simulink model "Main"  (R2025a)
settings: Solver=VariableStepAuto  StartTime=0.0  StopTime=inf  RelTol=1e-3
libraries: simulink x20, dspstat3 x10, simulink_extras x5, fuzblock x2
settings Model: Creator=felix  LastModifiedBy=lobakkang

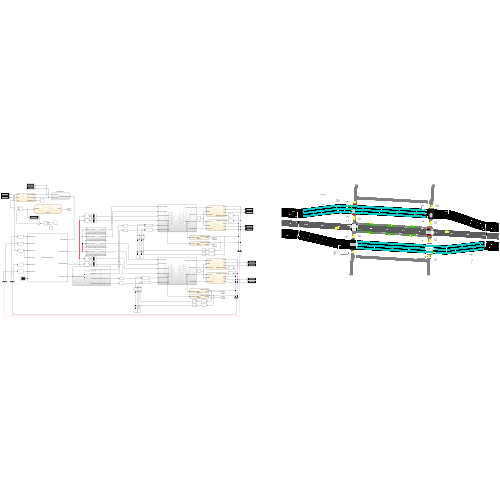
[thumbnail: Simulink's stored preview of the top-level diagram]
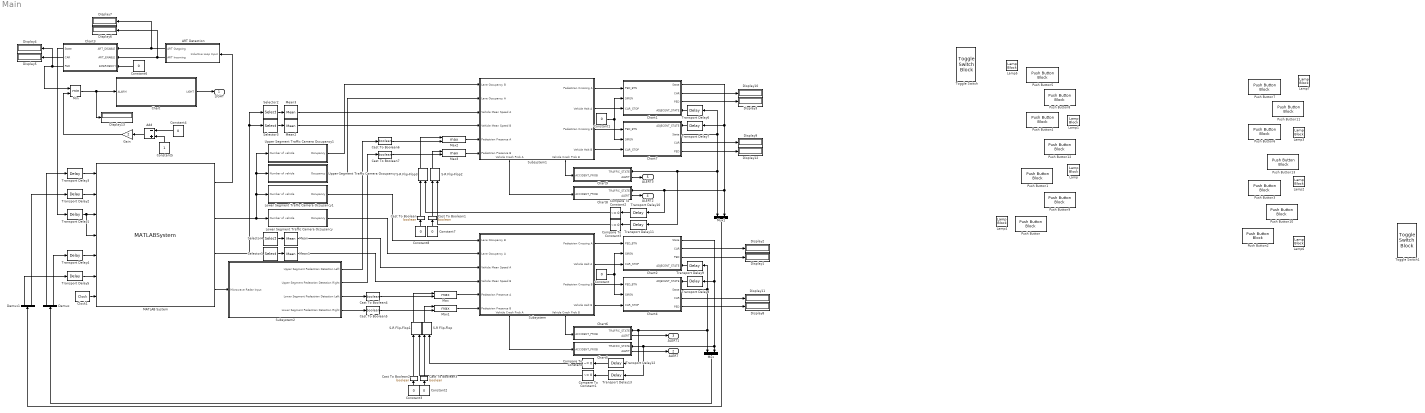
== system Main ==
  ART Detection : Subsystem
  Add : Sum  Inputs=-+
  Cast To Boolean{,1..7} (8 alike) : DataTypeConversion  OutDataTypeStr=boolean  SaturateOnIntegerOverflow=off  RndMeth=Floor
  Chart : Stateflow chart  TreatAsAtomicUnit=on
  Chart1 : Stateflow chart  TreatAsAtomicUnit=on
      settings: PortSchema="{\"entries\":[{\"content\":{\"sides\":[{\"content\":{\"connectorIds\":[\"In1\",\"In2\",\"In3\"]},\"type\":\"ConnectorPlacement.EquallySpacedRectSide\",\"uuid\":\"b25f2922-e8d8-447c-9fde-0a87dc56ab76\"},{\"content\":{\"connectorIds\":[\"Out1\",\"Out2\",\"Out3\",\"In4\"],\"side\":\"RIGHT\"},\"type\":\"ConnectorPlacement.EquallySpacedRectSide\",\"uuid\":\"421829cc-50ad-4948-b5ba-34d182ed9193\"},{\"content\":{\"side\":\"TOP\"},\"type\":\"ConnectorPlacement.EquallySpacedRectSide\",\"uuid\":\"15dcb3c0-9d0d-47c7-88ca-53369059b405\"},{\"content\":{\"side\":\"BOTTOM\"},\"type\":\"ConnectorPlacement.EquallySpacedRectSide\",\"uuid\":\"532ca745-839c-4cfc-92a4-9e4b119a98df\"}]},\"type\":\"ConnectorPlacement.EquallySpacedConnector\",\"uuid\":\"2a59643b-3d5f-42d6-a12d-4f5ba76c6b25\"}],\"packageUris\":[\"http://schema.mathworks.com/mf0/Connector/R2020b\"],\"version\":\"1.0\"}"
  Chart2 : Stateflow chart  TreatAsAtomicUnit=on
      settings: PortSchema="{\"entries\":[{\"content\":{\"sides\":[{\"content\":{\"connectorIds\":[\"In1\",\"In2\",\"In3\"]},\"type\":\"ConnectorPlacement.EquallySpacedRectSide\",\"uuid\":\"b25f2922-e8d8-447c-9fde-0a87dc56ab76\"},{\"content\":{\"connectorIds\":[\"Out1\",\"Out2\",\"Out3\",\"In4\"],\"side\":\"RIGHT\"},\"type\":\"ConnectorPlacement.EquallySpacedRectSide\",\"uuid\":\"421829cc-50ad-4948-b5ba-34d182ed9193\"},{\"content\":{\"side\":\"TOP\"},\"type\":\"ConnectorPlacement.EquallySpacedRectSide\",\"uuid\":\"15dcb3c0-9d0d-47c7-88ca-53369059b405\"},{\"content\":{\"side\":\"BOTTOM\"},\"type\":\"ConnectorPlacement.EquallySpacedRectSide\",\"uuid\":\"532ca745-839c-4cfc-92a4-9e4b119a98df\"}]},\"type\":\"ConnectorPlacement.EquallySpacedConnector\",\"uuid\":\"2a59643b-3d5f-42d6-a12d-4f5ba76c6b25\"}],\"packageUris\":[\"http://schema.mathworks.com/mf0/Connector/R2020b\"],\"version\":\"1.0\"}"
  Chart3 : Stateflow chart  TreatAsAtomicUnit=on
  Chart4 : Stateflow chart  TreatAsAtomicUnit=on
      settings: PortSchema="{\"entries\":[{\"content\":{\"sides\":[{\"content\":{\"connectorIds\":[\"In1\",\"In2\",\"In3\"]},\"type\":\"ConnectorPlacement.EquallySpacedRectSide\",\"uuid\":\"b25f2922-e8d8-447c-9fde-0a87dc56ab76\"},{\"content\":{\"connectorIds\":[\"In4\",\"Out1\",\"Out2\",\"Out3\"],\"side\":\"RIGHT\"},\"type\":\"ConnectorPlacement.EquallySpacedRectSide\",\"uuid\":\"421829cc-50ad-4948-b5ba-34d182ed9193\"},{\"content\":{\"side\":\"TOP\"},\"type\":\"ConnectorPlacement.EquallySpacedRectSide\",\"uuid\":\"15dcb3c0-9d0d-47c7-88ca-53369059b405\"},{\"content\":{\"side\":\"BOTTOM\"},\"type\":\"ConnectorPlacement.EquallySpacedRectSide\",\"uuid\":\"532ca745-839c-4cfc-92a4-9e4b119a98df\"}]},\"type\":\"ConnectorPlacement.EquallySpacedConnector\",\"uuid\":\"2a59643b-3d5f-42d6-a12d-4f5ba76c6b25\"}],\"packageUris\":[\"http://schema.mathworks.com/mf0/Connector/R2020b\"],\"version\":\"1.0\"}"
  Chart5 : Stateflow chart  TreatAsAtomicUnit=on
      settings: PortSchema="{\"entries\":[{\"content\":{\"sides\":[{\"content\":{\"connectorIds\":[\"In1\"]},\"type\":\"ConnectorPlacement.EquallySpacedRectSide\",\"uuid\":\"608d7dae-9529-4484-b16a-7c3c809a7af0\"},{\"content\":{\"connectorIds\":[\"In2\",\"Out1\"],\"side\":\"RIGHT\"},\"type\":\"ConnectorPlacement.EquallySpacedRectSide\",\"uuid\":\"13cec86d-a091-47ca-8c4c-06ad3ff59467\"},{\"content\":{\"side\":\"TOP\"},\"type\":\"ConnectorPlacement.EquallySpacedRectSide\",\"uuid\":\"91446a41-bf15-447e-8e76-a1311523585e\"}]},\"type\":\"ConnectorPlacement.EquallySpacedConnector\",\"uuid\":\"2a449cf7-a9fb-45d9-8ab4-45d23c1a1ddf\"}],\"packageUris\":[\"http://schema.mathworks.com/mf0/Connector/R2020b\"],\"version\":\"1.0\"}"
  Chart6 : Stateflow chart  TreatAsAtomicUnit=on
      settings: PortSchema="{\"entries\":[{\"content\":{\"sides\":[{\"content\":{\"connectorIds\":[\"In1\"]},\"type\":\"ConnectorPlacement.EquallySpacedRectSide\",\"uuid\":\"608d7dae-9529-4484-b16a-7c3c809a7af0\"},{\"content\":{\"connectorIds\":[\"In2\",\"Out1\"],\"side\":\"RIGHT\"},\"type\":\"ConnectorPlacement.EquallySpacedRectSide\",\"uuid\":\"13cec86d-a091-47ca-8c4c-06ad3ff59467\"},{\"content\":{\"side\":\"TOP\"},\"type\":\"ConnectorPlacement.EquallySpacedRectSide\",\"uuid\":\"91446a41-bf15-447e-8e76-a1311523585e\"}]},\"type\":\"ConnectorPlacement.EquallySpacedConnector\",\"uuid\":\"2a449cf7-a9fb-45d9-8ab4-45d23c1a1ddf\"}],\"packageUris\":[\"http://schema.mathworks.com/mf0/Connector/R2020b\"],\"version\":\"1.0\"}"
  Chart7 : Stateflow chart  TreatAsAtomicUnit=on
      settings: PortSchema="{\"entries\":[{\"content\":{\"sides\":[{\"content\":{\"connectorIds\":[\"In1\",\"In2\",\"In3\"]},\"type\":\"ConnectorPlacement.EquallySpacedRectSide\",\"uuid\":\"b25f2922-e8d8-447c-9fde-0a87dc56ab76\"},{\"content\":{\"connectorIds\":[\"In4\",\"Out1\",\"Out2\",\"Out3\"],\"side\":\"RIGHT\"},\"type\":\"ConnectorPlacement.EquallySpacedRectSide\",\"uuid\":\"421829cc-50ad-4948-b5ba-34d182ed9193\"},{\"content\":{\"side\":\"TOP\"},\"type\":\"ConnectorPlacement.EquallySpacedRectSide\",\"uuid\":\"15dcb3c0-9d0d-47c7-88ca-53369059b405\"},{\"content\":{\"side\":\"BOTTOM\"},\"type\":\"ConnectorPlacement.EquallySpacedRectSide\",\"uuid\":\"532ca745-839c-4cfc-92a4-9e4b119a98df\"}]},\"type\":\"ConnectorPlacement.EquallySpacedConnector\",\"uuid\":\"2a59643b-3d5f-42d6-a12d-4f5ba76c6b25\"}],\"packageUris\":[\"http://schema.mathworks.com/mf0/Connector/R2020b\"],\"version\":\"1.0\"}"
  Chart8 : Stateflow chart  TreatAsAtomicUnit=on
      settings: PortSchema="{\"entries\":[{\"content\":{\"sides\":[{\"content\":{\"connectorIds\":[\"In1\"]},\"type\":\"ConnectorPlacement.EquallySpacedRectSide\",\"uuid\":\"608d7dae-9529-4484-b16a-7c3c809a7af0\"},{\"content\":{\"connectorIds\":[\"In2\",\"Out1\"],\"side\":\"RIGHT\"},\"type\":\"ConnectorPlacement.EquallySpacedRectSide\",\"uuid\":\"13cec86d-a091-47ca-8c4c-06ad3ff59467\"},{\"content\":{\"side\":\"TOP\"},\"type\":\"ConnectorPlacement.EquallySpacedRectSide\",\"uuid\":\"91446a41-bf15-447e-8e76-a1311523585e\"}]},\"type\":\"ConnectorPlacement.EquallySpacedConnector\",\"uuid\":\"2a449cf7-a9fb-45d9-8ab4-45d23c1a1ddf\"}],\"packageUris\":[\"http://schema.mathworks.com/mf0/Connector/R2020b\"],\"version\":\"1.0\"}"
  Chart9 : Stateflow chart  TreatAsAtomicUnit=on
      settings: PortSchema="{\"entries\":[{\"content\":{\"sides\":[{\"content\":{\"connectorIds\":[\"In1\"]},\"type\":\"ConnectorPlacement.EquallySpacedRectSide\",\"uuid\":\"608d7dae-9529-4484-b16a-7c3c809a7af0\"},{\"content\":{\"connectorIds\":[\"In2\",\"Out1\"],\"side\":\"RIGHT\"},\"type\":\"ConnectorPlacement.EquallySpacedRectSide\",\"uuid\":\"13cec86d-a091-47ca-8c4c-06ad3ff59467\"},{\"content\":{\"side\":\"TOP\"},\"type\":\"ConnectorPlacement.EquallySpacedRectSide\",\"uuid\":\"91446a41-bf15-447e-8e76-a1311523585e\"}]},\"type\":\"ConnectorPlacement.EquallySpacedConnector\",\"uuid\":\"2a449cf7-a9fb-45d9-8ab4-45d23c1a1ddf\"}],\"packageUris\":[\"http://schema.mathworks.com/mf0/Connector/R2020b\"],\"version\":\"1.0\"}"
  Clock1 : simulink_extras/Flip Flops/Clock  period=1
  Compare To Constant{,1..3} (4 alike) : simulink/Logic and Bit Operations/Compare To Constant  relop=~=  const=0  OutDataTypeStr=boolean
  Constant{,1..4,6..8} (8 alike) : Constant  Value=0
  Constant5 : Constant
  Demux : Demux  Outputs=2
  Demux1 : Demux  Outputs=2
  Display{1..13} (13 alike) : Display
  Gain : Gain  Gain=2
  Lamp{,1..7} (8 alike) : LampBlock  LabelPosition=Hide  DefaultColor=[192.0, 192.0, 192.0]
  Lower Segment Traffic Camera Occupancy : Subsystem
  Lower Segment Traffic Camera Occupancy1 : Subsystem
  MATLAB System : MATLABSystem  System=TrafficSimulationSystem  Host=127.0.0.1  Port=55000  NumDetectors=4  NumInstantLoops=8  NumAreaDetectors=18  NumTrafficLights=6  SimulateUsing=Interpreted execution
      mask Type: TrafficSimulationSystem
  Max{,1..3} (4 alike) : MinMax  Function=max  Inputs=2
  Mean{,1..3} (4 alike) : dspstat3/Mean  run=off  InputProcessing=Columns as channels (frame based)  reset_popup=None  directionMode=Each column  dimension=1  roiEnable=off  roiType=Rectangles  roiPortion=Entire ROI  roiOutput=Individual statistics for each ROI  roiFlag=off  roundingMode=Floor  overflowMode=off  outputDataTypeStr=Inherit: Same as accumulator  outputMin=[]  outputMax=[]  outputLastDataTypeStr=Inherit: Same as accumulator
  Min : MinMax  Inputs=2
  Mux : Mux  Inputs=2
  Mux1 : Mux  Inputs=2
  Push Button{,1..5,7} (7 alike) : PushButtonBlock  IconOnColor=[0.0, 0.39215686274509803, 0.0]  IconOffColor=[0.0, 1.0, 0.0]  OffValue=0.000000
  Push Button{8..12} (5 alike) : PushButtonBlock  ButtonType=Latch  IconOnColor=[0.0, 0.39215686274509803, 0.0]  IconOffColor=[0.0, 1.0, 0.0]  OffValue=0.000000
  Push Button13 : PushButtonBlock  ButtonType=Latch  IconOnColor=[0.0, 0.39215686274509803, 0.0]  IconOffColor=[0.0, 1.0, 0.0]  OffValue=1.000000
  Push Button6 : PushButtonBlock  IconOnColor=[0.0, 0.39215686274509803, 0.0]  IconOffColor=[0.0, 1.0, 0.0]
  S-R Flip-Flop{,1..3} (4 alike) : simulink_extras/Flip Flops/S-R Flip-Flop  initial_condition=0
  Selector1 : Selector  IndexMode=Zero-based  InputPortWidth=18  IndexOptions=Index vector (dialog)  Indices=[6 7 8 9 10 11]  OutputSizes=1
  Selector2 : Selector  IndexMode=Zero-based  InputPortWidth=18  IndexOptions=Index vector (dialog)  Indices=[0 1 2 3 4 5]  OutputSizes=1
  Selector3 : Selector  IndexMode=Zero-based  InputPortWidth=18  IndexOptions=Index vector (dialog)  Indices=[12 13 15]  OutputSizes=1
  Selector4 : Selector  IndexMode=Zero-based  InputPortWidth=18  IndexOptions=Index vector (dialog)  Indices=[12 13 15]  OutputSizes=1
  Subsystem : Subsystem
      settings: PortSchema="{\"entries\":[{\"content\":{\"sides\":[{\"content\":{\"connectorIds\":[\"In1\",\"In2\",\"In3\",\"In4\",\"In5\",\"In6\"]},\"type\":\"ConnectorPlacement.EquallySpacedRectSide\",\"uuid\":\"53827b3a-c46a-4204-840d-e600012fe27f\"},{\"content\":{\"connectorIds\":[\"Out1\",\"Out2\",\"Out3\",\"Out4\"],\"side\":\"RIGHT\"},\"type\":\"ConnectorPlacement.EquallySpacedRectSide\",\"uuid\":\"cf707ced-ebab-43ca-9818-f6d8c721fe53\"},{\"content\":{\"side\":\"TOP\"},\"type\":\"ConnectorPlacement.EquallySpacedRectSide\",\"uuid\":\"16603e90-0a57-45b5-8379-ce405130782b\"},{\"content\":{\"connectorIds\":[\"Out5\",\"Out6\"],\"side\":\"BOTTOM\"},\"type\":\"ConnectorPlacement.EquallySpacedRectSide\",\"uuid\":\"f45158f6-4a74-4bd2-afbf-3c8c1bc11bef\"}]},\"type\":\"ConnectorPlacement.EquallySpacedConnector\",\"uuid\":\"52f23845-946f-443f-b18c-f1eea4db6dbd\"}],\"packageUris\":[\"http://schema.mathworks.com/mf0/Connector/R2020b\"],\"version\":\"1.0\"}"
  Subsystem1 : Subsystem
      settings: PortSchema="{\"entries\":[{\"content\":{\"sides\":[{\"content\":{\"connectorIds\":[\"In1\",\"In2\",\"In3\",\"In4\",\"In5\",\"In6\"]},\"type\":\"ConnectorPlacement.EquallySpacedRectSide\",\"uuid\":\"53827b3a-c46a-4204-840d-e600012fe27f\"},{\"content\":{\"connectorIds\":[\"Out1\",\"Out2\",\"Out3\",\"Out4\"],\"side\":\"RIGHT\"},\"type\":\"ConnectorPlacement.EquallySpacedRectSide\",\"uuid\":\"cf707ced-ebab-43ca-9818-f6d8c721fe53\"},{\"content\":{\"side\":\"TOP\"},\"type\":\"ConnectorPlacement.EquallySpacedRectSide\",\"uuid\":\"16603e90-0a57-45b5-8379-ce405130782b\"},{\"content\":{\"connectorIds\":[\"Out5\",\"Out6\"],\"side\":\"BOTTOM\"},\"type\":\"ConnectorPlacement.EquallySpacedRectSide\",\"uuid\":\"f45158f6-4a74-4bd2-afbf-3c8c1bc11bef\"}]},\"type\":\"ConnectorPlacement.EquallySpacedConnector\",\"uuid\":\"52f23845-946f-443f-b18c-f1eea4db6dbd\"}],\"packageUris\":[\"http://schema.mathworks.com/mf0/Connector/R2020b\"],\"version\":\"1.0\"}"
  Subsystem2 : Subsystem
  Toggle Switch : ToggleSwitchBlock
  Toggle Switch1 : ToggleSwitchBlock
  Transport Delay{1..13} (13 alike) : TransportDelay
  Upper Segment Traffic Camera Occupancy : Subsystem
  Upper Segment Traffic Camera Occupancy1 : Subsystem
  LIGHT : Outport
  ALERT : Outport  Port=2
  ALERT1 : Outport  Port=3
  ALERT2 : Outport  Port=4
  ALERT3 : Outport  Port=5
  wires:
  Transport Delay3/1 -> MATLAB System/1
  Transport Delay2/1 -> MATLAB System/2
  Chart3/3(PED) -> Display4/1, Min/1
  Chart3/2(CAR) -> Display5/1
  Transport Delay1/1 -> MATLAB System/4, MATLAB System/3
  Constant/1 -> Chart2/2(SIREN), Chart4/2(SIREN)
  Chart/1(LIGHT) -> LIGHT/1
  Min/1 -> Display13/1, Chart/1(ALARM)
  Gain/1 -> Min/2
  Add/1 -> Gain/1
  Constant4/1 -> Add/1
  Constant5/1 -> Add/2
  Constant6/1 -> Chart3/3(EMERGENCY)
  Clock1/1 -> MATLAB System/7
  Chart3/1(State) -> Transport Delay1/1
  MATLAB System/4 -> Subsystem2/1(Microwave Radar Input)
  ART Detection/2(ART Incoming) -> Chart3/2(ART_ENABLE), Display6/1
  ART Detection/1(ART Outgoing) -> Display7/1, Chart3/1(ART_DISABLE)
  MATLAB System/1 -> ART Detection/1(Inductive Loop Input)
  MATLAB System/3 -> Selector1/1, Selector2/1, Selector3/1, Selector4/1
  Selector4/1 -> Mean/1
  Selector1/1 -> Mean1/1
  Transport Delay4/1 -> MATLAB System/5
  Chart6/1(ALERT) -> ALERT1/1
  Lower Segment Traffic Camera Occupancy1/1(Occupancy) -> Subsystem/1(Lane Occupancy B)
  Lower Segment Traffic Camera Occupancy/1(Occupancy) -> Subsystem/2(Lane Occupancy A)
  Mean/1 -> Subsystem/3(Vehicle Mean Speed A)
  Mean1/1 -> Subsystem/4(Vehicle Mean Speed B)
  Subsystem/1(Pedestrian Crossing A) -> Chart2/1(PED_BTN)
  Subsystem/2(Vehicle Halt A) -> Chart2/3(CAR_STOP)
  Subsystem/3(Pedestrian Crossing B) -> Chart4/1(PED_BTN)
  Subsystem/4(Vehicle Halt B) -> Chart4/3(CAR_STOP)
  Subsystem/5(Vehicle Crash Prob A) -> Chart5/1(ACCIDENT_PROB)
  Subsystem/6(Vehicle Crash Prob B) -> Chart6/1(ACCIDENT_PROB)
  Transport Delay5/1 -> MATLAB System/6
  Demux/2 -> Transport Delay4/1
  Demux/1 -> Transport Delay3/1
  Chart4/1(State) -> Transport Delay12/1, Chart6/2(TRAFFIC_STATE), Mux/1, Transport Delay9/1
  Chart2/1(State) -> Transport Delay13/1, Chart5/2(TRAFFIC_STATE), Mux/2, Transport Delay8/1
  Chart1/1(State) -> Transport Delay7/1, Transport Delay10/1, Chart8/2(TRAFFIC_STATE), Mux1/2
  Chart7/1(State) -> Transport Delay11/1, Chart9/2(TRAFFIC_STATE), Mux1/1, Transport Delay6/1
  Subsystem1/6(Vehicle Crash Prob B) -> Chart9/1(ACCIDENT_PROB)
  Subsystem1/4(Vehicle Halt B) -> Chart7/3(CAR_STOP)
  Chart9/1(ALERT) -> ALERT3/1
  Subsystem1/2(Vehicle Halt A) -> Chart1/3(CAR_STOP)
  Subsystem1/3(Pedestrian Crossing B) -> Chart7/1(PED_BTN)
  Constant1/1 -> Chart1/2(SIREN), Chart7/2(SIREN)
  Chart1/2(CAR) -> Display10/1
  Subsystem1/5(Vehicle Crash Prob A) -> Chart8/1(ACCIDENT_PROB)
  Subsystem1/1(Pedestrian Crossing A) -> Chart1/1(PED_BTN)
  Chart8/1(ALERT) -> ALERT2/1
  Chart7/3(PED) -> Display12/1
  Chart1/3(PED) -> Display3/1
  Chart7/2(CAR) -> Display9/1
  Mux/1 -> Demux/1
  Mux1/1 -> Demux1/1
  MATLAB System/2 -> Lower Segment Traffic Camera Occupancy1/1(Number of vehicle), Upper Segment Traffic Camera Occupancy1/1(Number of vehicle), Upper Segment Traffic Camera Occupancy/1(Number of vehicle), Lower Segment Traffic Camera Occupancy/1(Number of vehicle)
  Upper Segment Traffic Camera Occupancy/1(Occupancy) -> Subsystem1/2(Lane Occupancy A)
  Upper Segment Traffic Camera Occupancy1/1(Occupancy) -> Subsystem1/1(Lane Occupancy B)
  Selector2/1 -> Mean3/1
  Selector3/1 -> Mean2/1
  Demux1/2 -> Transport Delay2/1
  Demux1/1 -> Transport Delay5/1
  Mean3/1 -> Subsystem1/3(Vehicle Mean Speed A)
  Mean2/1 -> Subsystem1/4(Vehicle Mean Speed B)
  Chart2/2(CAR) -> Display2/1
  Chart2/3(PED) -> Display1/1
  Chart4/2(CAR) -> Display11/1
  Chart4/3(PED) -> Display8/1
  Transport Delay6/1 -> Chart1/4(ADJECENT_STATE)
  Transport Delay7/1 -> Chart7/4(ADJECENT_STATE)
  Transport Delay8/1 -> Chart4/4(ADJECENT_STATE)
  Transport Delay9/1 -> Chart2/4(ADJECENT_STATE)
  Max1/1 -> Subsystem/6(Pedestrian Presence B)
  Max/1 -> Subsystem/5(Pedestrian Presence A)
  Subsystem2/3(Lower Segment Pedestrian Detection Left) -> Cast To Boolean4/1
  Subsystem2/4(Lower Segment Pedestrian Detection Right) -> Cast To Boolean5/1
  Max3/1 -> Subsystem1/6(Pedestrian Presence B)
  Subsystem2/2(Upper Segment Pedestrian Detection Right) -> Cast To Boolean7/1
  Max2/1 -> Subsystem1/5(Pedestrian Presence A)
  Subsystem2/1(Upper Segment Pedestrian Detection Left) -> Cast To Boolean6/1
  Chart5/1(ALERT) -> ALERT/1
  Constant2/1 -> Cast To Boolean3/1
  S-R Flip-Flop/1 -> Max1/1
  Constant3/1 -> Cast To Boolean2/1
  S-R Flip-Flop1/1 -> Max/1
  Compare To Constant/1 -> S-R Flip-Flop/2
  Compare To Constant1/1 -> S-R Flip-Flop1/2
  Constant7/1 -> Cast To Boolean1/1
  Constant8/1 -> Cast To Boolean/1
  S-R Flip-Flop2/1 -> Max3/1
  S-R Flip-Flop3/1 -> Max2/1
  Compare To Constant3/1 -> S-R Flip-Flop2/2
  Compare To Constant2/1 -> S-R Flip-Flop3/2
  Cast To Boolean/1 -> S-R Flip-Flop3/1
  Cast To Boolean1/1 -> S-R Flip-Flop2/1
  Cast To Boolean3/1 -> S-R Flip-Flop/1
  Cast To Boolean2/1 -> S-R Flip-Flop1/1
  Cast To Boolean4/1 -> Max/2
  Cast To Boolean5/1 -> Max1/2
  Cast To Boolean6/1 -> Max2/2
  Cast To Boolean7/1 -> Max3/2
  Transport Delay10/1 -> Compare To Constant2/1
  Transport Delay11/1 -> Compare To Constant3/1
  Transport Delay13/1 -> Compare To Constant1/1
  Transport Delay12/1 -> Compare To Constant/1

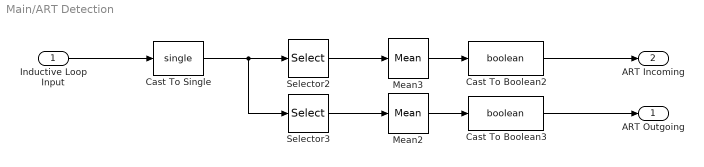
== system Main/ART Detection ==
  Inductive Loop Input : Inport
  Cast To Boolean2 : DataTypeConversion  OutDataTypeStr=boolean  SaturateOnIntegerOverflow=off  RndMeth=Floor
  Cast To Boolean3 : DataTypeConversion  OutDataTypeStr=boolean  SaturateOnIntegerOverflow=off  RndMeth=Floor
  Cast To Single : DataTypeConversion  OutDataTypeStr=single  SaturateOnIntegerOverflow=off  RndMeth=Floor
  Mean2 : dspstat3/Mean  run=off  InputProcessing=Columns as channels (frame based)  reset_popup=None  directionMode=Each column  dimension=1  roiEnable=off  roiType=Rectangles  roiPortion=Entire ROI  roiOutput=Individual statistics for each ROI  roiFlag=off  roundingMode=Floor  overflowMode=off  outputDataTypeStr=Inherit: Same as accumulator  outputMin=[]  outputMax=[]  outputLastDataTypeStr=Inherit: Same as accumulator
  Mean3 : dspstat3/Mean  run=off  InputProcessing=Columns as channels (frame based)  reset_popup=None  directionMode=Each column  dimension=1  roiEnable=off  roiType=Rectangles  roiPortion=Entire ROI  roiOutput=Individual statistics for each ROI  roiFlag=off  roundingMode=Floor  overflowMode=off  outputDataTypeStr=Inherit: Same as accumulator  outputMin=[]  outputMax=[]  outputLastDataTypeStr=Inherit: Same as accumulator
  Selector2 : Selector  InputPortWidth=4  IndexOptions=Index vector (dialog)  Indices=[3 2]  OutputSizes=1
  Selector3 : Selector  InputPortWidth=4  IndexOptions=Index vector (dialog)  Indices=[1 4]  OutputSizes=1
  ART Outgoing : Outport
  ART Incoming : Outport  Port=2
  wires:
  Mean2/1 -> Cast To Boolean3/1
  Mean3/1 -> Cast To Boolean2/1
  Cast To Single/1 -> Selector3/1, Selector2/1
  Selector3/1 -> Mean2/1
  Inductive Loop Input/1 -> Cast To Single/1
  Selector2/1 -> Mean3/1
  Cast To Boolean2/1 -> ART Incoming/1
  Cast To Boolean3/1 -> ART Outgoing/1

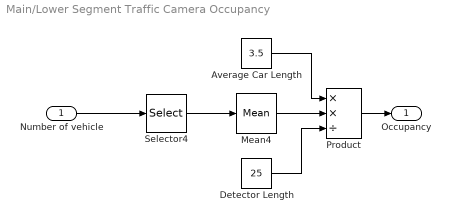
== system Main/Lower Segment Traffic Camera Occupancy ==
  Number of vehicle : Inport
  Average Car Length : Constant  Value=3.5
  Detector Length : Constant  Value=25
  Mean4 : dspstat3/Mean  run=off  InputProcessing=Columns as channels (frame based)  reset_popup=None  directionMode=Each column  dimension=1  roiEnable=off  roiType=Rectangles  roiPortion=Entire ROI  roiOutput=Individual statistics for each ROI  roiFlag=off  roundingMode=Floor  overflowMode=off  outputDataTypeStr=Inherit: Same as accumulator  outputMin=[]  outputMax=[]  outputLastDataTypeStr=Inherit: Same as accumulator
  Product : Product  Inputs=**/
  Selector4 : Selector  IndexMode=Zero-based  InputPortWidth=18  IndexOptions=Index vector (dialog)  Indices=[9 10 11 6 7 8]  OutputSizes=1
  Occupancy : Outport
  wires:
  Number of vehicle/1 -> Selector4/1
  Detector Length/1 -> Product/3
  Selector4/1 -> Mean4/1
  Mean4/1 -> Product/2
  Average Car Length/1 -> Product/1
  Product/1 -> Occupancy/1

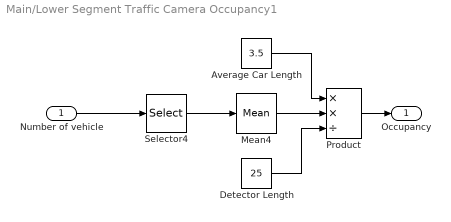
== system Main/Lower Segment Traffic Camera Occupancy1 ==
  Number of vehicle : Inport
  Average Car Length : Constant  Value=3.5
  Detector Length : Constant  Value=25
  Mean4 : dspstat3/Mean  run=off  InputProcessing=Columns as channels (frame based)  reset_popup=None  directionMode=Each column  dimension=1  roiEnable=off  roiType=Rectangles  roiPortion=Entire ROI  roiOutput=Individual statistics for each ROI  roiFlag=off  roundingMode=Floor  overflowMode=off  outputDataTypeStr=Inherit: Same as accumulator  outputMin=[]  outputMax=[]  outputLastDataTypeStr=Inherit: Same as accumulator
  Product : Product  Inputs=**/
  Selector4 : Selector  IndexMode=Zero-based  InputPortWidth=18  IndexOptions=Index vector (dialog)  Indices=[12 13 15]  OutputSizes=1
  Occupancy : Outport
  wires:
  Number of vehicle/1 -> Selector4/1
  Detector Length/1 -> Product/3
  Selector4/1 -> Mean4/1
  Mean4/1 -> Product/2
  Average Car Length/1 -> Product/1
  Product/1 -> Occupancy/1

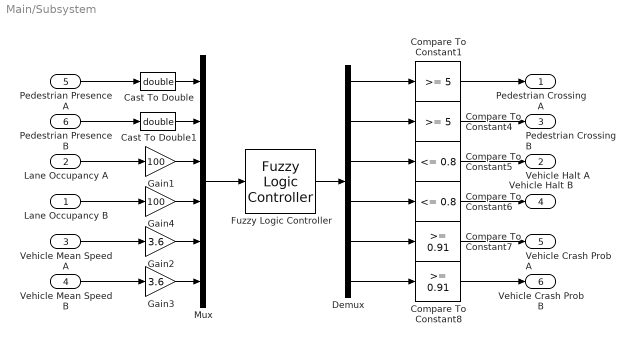
== system Main/Subsystem ==
  Lane Occupancy B : Inport
  Lane Occupancy A : Inport  Port=2
  Vehicle Mean Speed A : Inport  Port=3
  Vehicle Mean Speed B : Inport  Port=4
  Pedestrian Presence A : Inport  Port=5
  Pedestrian Presence B : Inport  Port=6
  Cast To Double : DataTypeConversion  OutDataTypeStr=double  SaturateOnIntegerOverflow=off  RndMeth=Floor
  Cast To Double1 : DataTypeConversion  OutDataTypeStr=double  SaturateOnIntegerOverflow=off  RndMeth=Floor
  Compare To Constant1 : simulink/Logic and Bit Operations/Compare To Constant  relop=>=  const=5  OutDataTypeStr=uint8
  Compare To Constant4 : simulink/Logic and Bit Operations/Compare To Constant  relop=>=  const=5  OutDataTypeStr=uint8
  Compare To Constant5 : simulink/Logic and Bit Operations/Compare To Constant  relop=<=  const=0.8  OutDataTypeStr=uint8
  Compare To Constant6 : simulink/Logic and Bit Operations/Compare To Constant  relop=<=  const=0.8  OutDataTypeStr=uint8
  Compare To Constant7 : simulink/Logic and Bit Operations/Compare To Constant  relop=>=  const=0.91  OutDataTypeStr=uint8
  Compare To Constant8 : simulink/Logic and Bit Operations/Compare To Constant  relop=>=  const=0.91  OutDataTypeStr=uint8
  Demux : Demux  Outputs=6
  Fuzzy Logic Controller : fuzblock/Fuzzy Logic  Controller  FIS='PedestrianController.fis'  OutputSampleNumber=101  DataType=double  UseLookupTable=off  NumBreakpoints=10  FuzzifiedInputs=off  RuleFiringStrengths=off  RuleOutputs=off  AggregatedOutputs=off  SimulateUsing=Code generation  OutOfRangeInputValueMessage=warning  NoRuleFiredMessage=warning  EmptyOutputFuzzySetMessage=warning
  Gain1 : Gain  Gain=100
  Gain2 : Gain  Gain=3.6
  Gain3 : Gain  Gain=3.6
  Gain4 : Gain  Gain=100
  Mux : Mux  Inputs=6
  Pedestrian Crossing A : Outport
  Vehicle Halt A : Outport  Port=2
  Pedestrian Crossing B : Outport  Port=3
  Vehicle Halt B : Outport  Port=4
  Vehicle Crash Prob A : Outport  Port=5
  Vehicle Crash Prob B : Outport  Port=6
  wires:
  Gain3/1 -> Mux/6
  Mux/1 -> Fuzzy Logic Controller/1
  Demux/1 -> Compare To Constant1/1
  Vehicle Mean Speed A/1 -> Gain2/1
  Demux/5 -> Compare To Constant7/1
  Fuzzy Logic Controller/1 -> Demux/1
  Demux/6 -> Compare To Constant8/1
  Cast To Double1/1 -> Mux/2
  Demux/4 -> Compare To Constant6/1
  Demux/3 -> Compare To Constant5/1
  Gain1/1 -> Mux/3
  Demux/2 -> Compare To Constant4/1
  Gain4/1 -> Mux/4
  Cast To Double/1 -> Mux/1
  Gain2/1 -> Mux/5
  Compare To Constant7/1 -> Vehicle Crash Prob A/1
  Pedestrian Presence B/1 -> Cast To Double1/1
  Pedestrian Presence A/1 -> Cast To Double/1
  Compare To Constant6/1 -> Vehicle Halt B/1
  Lane Occupancy A/1 -> Gain1/1
  Compare To Constant4/1 -> Pedestrian Crossing B/1
  Lane Occupancy B/1 -> Gain4/1
  Vehicle Mean Speed B/1 -> Gain3/1
  Compare To Constant8/1 -> Vehicle Crash Prob B/1
  Compare To Constant5/1 -> Vehicle Halt A/1
  Compare To Constant1/1 -> Pedestrian Crossing A/1

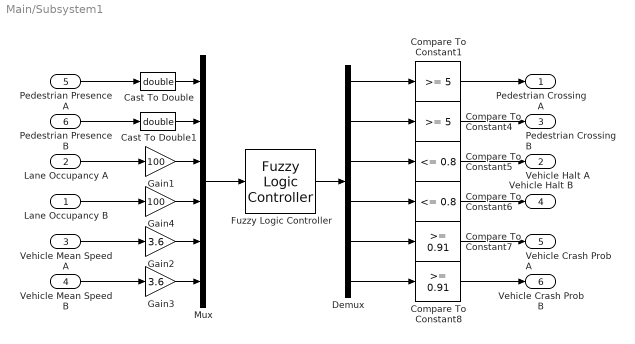
== system Main/Subsystem1 ==
  Lane Occupancy B : Inport
  Lane Occupancy A : Inport  Port=2
  Vehicle Mean Speed A : Inport  Port=3
  Vehicle Mean Speed B : Inport  Port=4
  Pedestrian Presence A : Inport  Port=5
  Pedestrian Presence B : Inport  Port=6
  Cast To Double : DataTypeConversion  OutDataTypeStr=double  SaturateOnIntegerOverflow=off  RndMeth=Floor
  Cast To Double1 : DataTypeConversion  OutDataTypeStr=double  SaturateOnIntegerOverflow=off  RndMeth=Floor
  Compare To Constant1 : simulink/Logic and Bit Operations/Compare To Constant  relop=>=  const=5  OutDataTypeStr=uint8
  Compare To Constant4 : simulink/Logic and Bit Operations/Compare To Constant  relop=>=  const=5  OutDataTypeStr=uint8
  Compare To Constant5 : simulink/Logic and Bit Operations/Compare To Constant  relop=<=  const=0.8  OutDataTypeStr=uint8
  Compare To Constant6 : simulink/Logic and Bit Operations/Compare To Constant  relop=<=  const=0.8  OutDataTypeStr=uint8
  Compare To Constant7 : simulink/Logic and Bit Operations/Compare To Constant  relop=>=  const=0.91  OutDataTypeStr=uint8
  Compare To Constant8 : simulink/Logic and Bit Operations/Compare To Constant  relop=>=  const=0.91  OutDataTypeStr=uint8
  Demux : Demux  Outputs=6
  Fuzzy Logic Controller : fuzblock/Fuzzy Logic  Controller  FIS='PedestrianController.fis'  OutputSampleNumber=101  DataType=double  UseLookupTable=off  NumBreakpoints=10  FuzzifiedInputs=off  RuleFiringStrengths=off  RuleOutputs=off  AggregatedOutputs=off  SimulateUsing=Code generation  OutOfRangeInputValueMessage=warning  NoRuleFiredMessage=warning  EmptyOutputFuzzySetMessage=warning
  Gain1 : Gain  Gain=100
  Gain2 : Gain  Gain=3.6
  Gain3 : Gain  Gain=3.6
  Gain4 : Gain  Gain=100
  Mux : Mux  Inputs=6
  Pedestrian Crossing A : Outport
  Vehicle Halt A : Outport  Port=2
  Pedestrian Crossing B : Outport  Port=3
  Vehicle Halt B : Outport  Port=4
  Vehicle Crash Prob A : Outport  Port=5
  Vehicle Crash Prob B : Outport  Port=6
  wires:
  Gain3/1 -> Mux/6
  Mux/1 -> Fuzzy Logic Controller/1
  Demux/1 -> Compare To Constant1/1
  Vehicle Mean Speed A/1 -> Gain2/1
  Demux/5 -> Compare To Constant7/1
  Fuzzy Logic Controller/1 -> Demux/1
  Demux/6 -> Compare To Constant8/1
  Cast To Double1/1 -> Mux/2
  Demux/4 -> Compare To Constant6/1
  Demux/3 -> Compare To Constant5/1
  Gain1/1 -> Mux/3
  Demux/2 -> Compare To Constant4/1
  Gain4/1 -> Mux/4
  Cast To Double/1 -> Mux/1
  Gain2/1 -> Mux/5
  Compare To Constant7/1 -> Vehicle Crash Prob A/1
  Pedestrian Presence B/1 -> Cast To Double1/1
  Pedestrian Presence A/1 -> Cast To Double/1
  Compare To Constant6/1 -> Vehicle Halt B/1
  Lane Occupancy A/1 -> Gain1/1
  Compare To Constant4/1 -> Pedestrian Crossing B/1
  Lane Occupancy B/1 -> Gain4/1
  Vehicle Mean Speed B/1 -> Gain3/1
  Compare To Constant8/1 -> Vehicle Crash Prob B/1
  Compare To Constant5/1 -> Vehicle Halt A/1
  Compare To Constant1/1 -> Pedestrian Crossing A/1

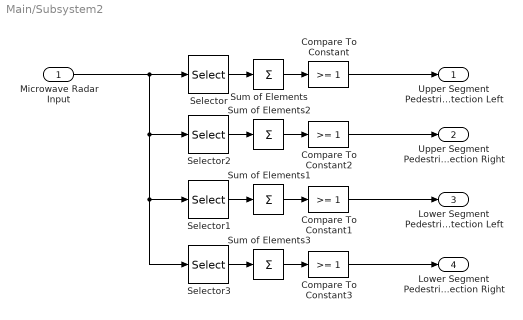
== system Main/Subsystem2 ==
  Microwave Radar Input : Inport
  Compare To Constant{,1..3} (4 alike) : simulink/Logic and Bit Operations/Compare To Constant  relop=>=  const=1  OutDataTypeStr=uint8
  Selector : Selector  InputPortWidth=8  IndexOptions=Index vector (dialog)  Indices=[6 7]  OutputSizes=1
  Selector1 : Selector  InputPortWidth=8  IndexOptions=Index vector (dialog)  Indices=[1 4]  OutputSizes=1
  Selector2 : Selector  InputPortWidth=8  IndexOptions=Index vector (dialog)  Indices=[5 8]  OutputSizes=1
  Selector3 : Selector  InputPortWidth=8  IndexOptions=Index vector (dialog)  Indices=[2 3]  OutputSizes=1
  Sum of Elements{,1..3} (4 alike) : Sum  Inputs=+
  Upper Segment Pedestrian Detection Left : Outport
  Upper Segment Pedestrian Detection Right : Outport  Port=2
  Lower Segment Pedestrian Detection Left : Outport  Port=3
  Lower Segment Pedestrian Detection Right : Outport  Port=4
  wires:
  Compare To Constant1/1 -> Lower Segment Pedestrian Detection Left/1
  Compare To Constant/1 -> Upper Segment Pedestrian Detection Left/1
  Sum of Elements/1 -> Compare To Constant/1
  Selector/1 -> Sum of Elements/1
  Selector1/1 -> Sum of Elements1/1
  Sum of Elements1/1 -> Compare To Constant1/1
  Compare To Constant2/1 -> Upper Segment Pedestrian Detection Right/1
  Selector2/1 -> Sum of Elements2/1
  Sum of Elements2/1 -> Compare To Constant2/1
  Selector3/1 -> Sum of Elements3/1
  Compare To Constant3/1 -> Lower Segment Pedestrian Detection Right/1
  Sum of Elements3/1 -> Compare To Constant3/1
  Microwave Radar Input/1 -> Selector/1, Selector2/1, Selector3/1, Selector1/1

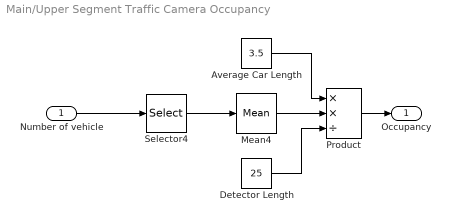
== system Main/Upper Segment Traffic Camera Occupancy ==
  Number of vehicle : Inport
  Average Car Length : Constant  Value=3.5
  Detector Length : Constant  Value=25
  Mean4 : dspstat3/Mean  run=off  InputProcessing=Columns as channels (frame based)  reset_popup=None  directionMode=Each column  dimension=1  roiEnable=off  roiType=Rectangles  roiPortion=Entire ROI  roiOutput=Individual statistics for each ROI  roiFlag=off  roundingMode=Floor  overflowMode=off  outputDataTypeStr=Inherit: Same as accumulator  outputMin=[]  outputMax=[]  outputLastDataTypeStr=Inherit: Same as accumulator
  Product : Product  Inputs=**/
  Selector4 : Selector  IndexMode=Zero-based  InputPortWidth=18  IndexOptions=Index vector (dialog)  Indices=[0 1 2 3 4 5]  OutputSizes=1
  Occupancy : Outport
  wires:
  Number of vehicle/1 -> Selector4/1
  Detector Length/1 -> Product/3
  Selector4/1 -> Mean4/1
  Mean4/1 -> Product/2
  Average Car Length/1 -> Product/1
  Product/1 -> Occupancy/1

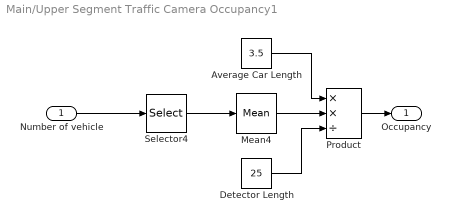
== system Main/Upper Segment Traffic Camera Occupancy1 ==
  Number of vehicle : Inport
  Average Car Length : Constant  Value=3.5
  Detector Length : Constant  Value=25
  Mean4 : dspstat3/Mean  run=off  InputProcessing=Columns as channels (frame based)  reset_popup=None  directionMode=Each column  dimension=1  roiEnable=off  roiType=Rectangles  roiPortion=Entire ROI  roiOutput=Individual statistics for each ROI  roiFlag=off  roundingMode=Floor  overflowMode=off  outputDataTypeStr=Inherit: Same as accumulator  outputMin=[]  outputMax=[]  outputLastDataTypeStr=Inherit: Same as accumulator
  Product : Product  Inputs=**/
  Selector4 : Selector  IndexMode=Zero-based  InputPortWidth=18  IndexOptions=Index vector (dialog)  Indices=[14 16 17]  OutputSizes=1
  Occupancy : Outport
  wires:
  Number of vehicle/1 -> Selector4/1
  Detector Length/1 -> Product/3
  Selector4/1 -> Mean4/1
  Mean4/1 -> Product/2
  Average Car Length/1 -> Product/1
  Product/1 -> Occupancy/1

== stateflow chart Main/Chart ==
  settings: stateMachineType=MOORE_MACHINE  executeAtInitialization=1
  state IDLE
    LIGHT=1;
  state FLASH
    LIGHT=1;
  state FLASH2
    LIGHT=0;
  (default) -> IDLE
  FLASH -> IDLE [order 1] : [ALARM==2]
  IDLE -> FLASH : [ALARM==0]
  FLASH2 -> FLASH : [after(0.2, sec)]
  FLASH -> FLASH2 [order 2] : [after(0.2, sec)]
  data: LIGHT output double; ALARM input

== stateflow chart Main/Chart4 ==
  state CAR_GREEN
    entry:
    CAR=2;
    PED=0;
    State=0;
  state CAR_YELLOW
    entry:
    CAR=1;
    PED=0;
    State=1;
  state ALL_RED
    entry:
    CAR=0;
    PED=0;
    State=3;
  state PED_GREEN
    entry:
    CAR=0;
    PED=2;
    State=2;
  (default) -> CAR_GREEN
  CAR_GREEN -> CAR_GREEN [order 2] : [ADJECENT_STATE!=0]
  CAR_GREEN -> CAR_YELLOW [order 3] : [PED_BTN==1&&ADJECENT_STATE==0&&SIREN==0&&after(30, sec)]
  CAR_GREEN -> PED_GREEN [order 1] : [ADJECENT_STATE==2]
  PED_GREEN -> CAR_GREEN [order 1] : [SIREN==1]
  ALL_RED -> CAR_GREEN : [after(3, sec)]
  CAR_YELLOW -> PED_GREEN : [after(8, sec)||(after(2, sec)&&CAR_STOP==1)]
  PED_GREEN -> ALL_RED [order 2] : [PED_BTN==0&&after(10, sec)]
  data: State output double; CAR output double; PED output double; PED_BTN input; SIREN input; CAR_STOP input; ADJECENT_STATE input

== stateflow chart Main/Chart5 ==
  settings: stateMachineType=MOORE_MACHINE  executeAtInitialization=1
  state NORMAL
    ALERT=0;
  state ACCIDENT
    ALERT=1;
  (default) -> NORMAL
  NORMAL -> NORMAL [order 1] : [TRAFFIC_STATE!=0]
  NORMAL -> ACCIDENT [order 2] : [ACCIDENT_PROB==1&&TRAFFIC_STATE==0&&after(15, sec)]
  ACCIDENT -> NORMAL : [ACCIDENT_PROB==0&&after(10, sec)]
  data: ALERT output double; ACCIDENT_PROB input; TRAFFIC_STATE input

== stateflow chart Main/Chart6 ==
  settings: stateMachineType=MOORE_MACHINE  executeAtInitialization=1
  state NORMAL
    ALERT=0;
  state ACCIDENT
    ALERT=1;
  (default) -> NORMAL
  NORMAL -> NORMAL [order 1] : [TRAFFIC_STATE!=0]
  NORMAL -> ACCIDENT [order 2] : [ACCIDENT_PROB==1&&TRAFFIC_STATE==0&&after(15, sec)]
  ACCIDENT -> NORMAL : [ACCIDENT_PROB==0&&after(10, sec)]
  data: ALERT output double; ACCIDENT_PROB input; TRAFFIC_STATE input

== stateflow chart Main/Chart7 ==
  state CAR_GREEN
    entry:
    CAR=2;
    PED=0;
    State=0;
  state CAR_YELLOW
    entry:
    CAR=1;
    PED=0;
    State=1;
  state ALL_RED
    entry:
    CAR=0;
    PED=0;
    State=3;
  state PED_GREEN
    entry:
    CAR=0;
    PED=2;
    State=2;
  (default) -> CAR_GREEN
  CAR_GREEN -> CAR_GREEN [order 2] : [ADJECENT_STATE!=0]
  CAR_GREEN -> CAR_YELLOW [order 3] : [PED_BTN==1&&ADJECENT_STATE==0&&SIREN==0&&after(30, sec)]
  CAR_GREEN -> PED_GREEN [order 1] : [ADJECENT_STATE==2]
  PED_GREEN -> CAR_GREEN [order 1] : [SIREN==1]
  ALL_RED -> CAR_GREEN : [after(3, sec)]
  CAR_YELLOW -> PED_GREEN : [after(8, sec)||(after(2, sec)&&CAR_STOP==1)]
  PED_GREEN -> ALL_RED [order 2] : [PED_BTN==0&&after(10, sec)]
  data: State output double; CAR output double; PED output double; PED_BTN input; SIREN input; CAR_STOP input; ADJECENT_STATE input

== stateflow chart Main/Chart8 ==
  settings: stateMachineType=MOORE_MACHINE  executeAtInitialization=1
  state NORMAL
    ALERT=0;
  state ACCIDENT
    ALERT=1;
  (default) -> NORMAL
  NORMAL -> NORMAL [order 1] : [TRAFFIC_STATE!=0]
  NORMAL -> ACCIDENT [order 2] : [ACCIDENT_PROB==1&&TRAFFIC_STATE==0&&after(15, sec)]
  ACCIDENT -> NORMAL : [ACCIDENT_PROB==0&&after(10, sec)]
  data: ALERT output double; ACCIDENT_PROB input; TRAFFIC_STATE input

== stateflow chart Main/Chart9 ==
  settings: stateMachineType=MOORE_MACHINE  executeAtInitialization=1
  state NORMAL
    ALERT=0;
  state ACCIDENT
    ALERT=1;
  (default) -> NORMAL
  NORMAL -> NORMAL [order 1] : [TRAFFIC_STATE!=0]
  NORMAL -> ACCIDENT [order 2] : [ACCIDENT_PROB==1&&TRAFFIC_STATE==0&&after(15, sec)]
  ACCIDENT -> NORMAL : [ACCIDENT_PROB==0&&after(10, sec)]
  data: ALERT output double; ACCIDENT_PROB input; TRAFFIC_STATE input

== stateflow chart Main/Chart1 ==
  state CAR_GREEN
    entry:
    CAR=2;
    PED=0;
    State=0;
  state CAR_YELLOW
    entry:
    CAR=1;
    PED=0;
    State=1;
  state ALL_RED
    entry:
    CAR=0;
    PED=0;
    State=3;
  state PED_GREEN
    entry:
    CAR=0;
    PED=2;
    State=2;
  (default) -> CAR_GREEN
  CAR_GREEN -> CAR_GREEN [order 1] : [ADJECENT_STATE!=0]
  CAR_GREEN -> CAR_YELLOW [order 2] : [PED_BTN==1&&ADJECENT_STATE==0&&SIREN==0&&after(30, sec)]
  PED_GREEN -> CAR_GREEN [order 1] : [SIREN==1]
  ALL_RED -> CAR_GREEN : [after(3, sec)]
  CAR_YELLOW -> PED_GREEN : [after(8, sec)||(after(2, sec)&&CAR_STOP==1)]
  PED_GREEN -> ALL_RED [order 2] : [PED_BTN==0&&after(10, sec)]
  data: State output double; CAR output double; PED output double; PED_BTN input; SIREN input; CAR_STOP input; ADJECENT_STATE input

== stateflow chart Main/Chart2 ==
  state CAR_GREEN
    entry:
    CAR=2;
    PED=0;
    State=0;
  state CAR_YELLOW
    entry:
    CAR=1;
    PED=0;
    State=1;
  state ALL_RED
    entry:
    CAR=0;
    PED=0;
    State=3;
  state PED_GREEN
    entry:
    CAR=0;
    PED=2;
    State=2;
  (default) -> CAR_GREEN
  CAR_GREEN -> CAR_GREEN [order 1] : [ADJECENT_STATE!=0]
  CAR_GREEN -> CAR_YELLOW [order 2] : [PED_BTN==1&&ADJECENT_STATE==0&&SIREN==0&&after(30, sec)]
  PED_GREEN -> CAR_GREEN [order 1] : [SIREN==1]
  ALL_RED -> CAR_GREEN : [after(3, sec)]
  CAR_YELLOW -> PED_GREEN : [after(8, sec)||(after(2, sec)&&CAR_STOP==1)]
  PED_GREEN -> ALL_RED [order 2] : [PED_BTN==0&&after(10, sec)]
  data: State output double; CAR output double; PED output double; PED_BTN input; SIREN input; CAR_STOP input; ADJECENT_STATE input

== stateflow chart Main/Chart3 ==
  state CAR_GREEN
    entry:
    CAR=2;
    PED=0;
    State=0;
  state CAR_YELLOW
    entry:
    CAR=1;
    PED=0;
    State=1;
  state ALL_RED
    entry:
    CAR=0;
    PED=0;
    State=3;
  state PED_GREEN
    entry:
    CAR=0;
    PED=2;
    State=2;
  CAR_GREEN -> CAR_YELLOW : [ART_DISABLE==1]
  ALL_RED -> CAR_GREEN : [after(0.1, sec)]
  CAR_YELLOW -> PED_GREEN : [after(2, sec)]
  (default) -> PED_GREEN
  PED_GREEN -> ALL_RED : [ART_ENABLE==1&&EMERGENCY==0]
  data: State output double; CAR output double; PED output double; ART_DISABLE input; ART_ENABLE input; EMERGENCY input
